simulink model "heli_q8_lab2_part1"  (R2020b)
settings: Solver=ode1  StartTime=0.0  StopTime=inf  FixedStep=0.002  RelTol=1e-3  EnableMultiTasking=on
PostLoadFcn:
  | qc_set_target_type(getConfigSet(bdroot, 'QUARC Default Target Configuration'));
values from neighbouring files (symbols this model uses):
  elev_const = 0.53    [init_heli_3_10_part_4.m]
  F_1 = [K_1(1,1) K_1(1,3) ... (first row only)    [init_heli_3_10_part_4.m]
  Joystick_gain_x = 1    [init_heli_3_10_part_4.m]
  Joystick_gain_y = -1    [init_heli_3_10_part_4.m]
  K_1 = lqr(A,B, Q_lqr, R_lqr)    [init_heli_3_10_part_4.m]
  V_s_0 = 7.77    [init_heli_3_10_part_4.m]
undefined symbols (not defined in the file or in its folder): HIL, qc_get_step_size, sigbuilder_block
libraries: quarc_library x4
settings Model: SimulationMode=external  ExtModeTrigDuration=5000  Creator=Rchan  LastModifiedBy=saavim
settings SolverCC: PositivePriorityOrder=on
settings DataIOCC: LimitDataPoints=on  SaveFormat=Array  SignalLoggingSaveFormat=ModelDataLogs  ReturnWorkspaceOutputs=off
settings OptimizationCC: ExpressionDepthLimit=2147483647  InitFltsAndDblsToZero=on  LifeSpan=inf
settings DebuggingCC: SaveWithParameterizedLinksMsg=none  UnderspecifiedInitializationDetection=Classic  MergeDetectMultiDrivingBlocksExec=none  SolverPrmCheckMsg=warning  MultiTaskDSMMsg=warning  MultiTaskCondExecSysMsg=none  FcnCallInpInsideContextMsg=warning  AllowSymbolicDim=off  StateNameClashWarn=warning  SFUnexpectedBacktrackingDiag=warning  SFNoUnconditionalDefaultTransitionDiag=warning  SFExecutionAtInitializationDiag=none  ArithmeticOperatorsInVariantConditions=warning
settings HardwareCC: ProdBitPerPointer=32  ProdBitPerSizeT=32  ProdBitPerPtrDiffT=32  ProdLargestAtomicFloat=None  ProdIntDivRoundTo=Undefined  ProdEndianess=Unspecified  ProdWordSize=32  ProdHWDeviceType=32-bit Generic
settings ModelReferenceCC: PropagateSignalLabelsOutOfModel=off
settings SFSimCC: SimUseLocalCustomCode=off  CustomCodeUndefinedFunction=UseInterfaceOnly
settings RTWCC: Description=QUARC Win64 Target  SystemTargetFile=quarc_win64.tlc  TemplateMakefile=quarc_default_tmf  RTWUseLocalCustomCode=off
settings CodeAppCC: StateflowObjectComments=on
settings GRTTargetCC: TargetLangStandard=C89/C90 (ANSI)  ParMdlRefBuildCompliant=off  CompOptLevelCompliant=off  CombineOutputUpdateFcns=off  MatFileLogging=off  GRTInterface=on  UseToolchainInfoCompliant=off  ExtMode=on  ExtModeMexFile=quarc_comm
settings ConfigComp: CovMetricSettings=dw  CovSaveCumulativeToWorkspaceVar=on  CovSaveSingleToWorkspaceVar=on  CovExternalEMLEnable=off  CovSFcnEnable=off

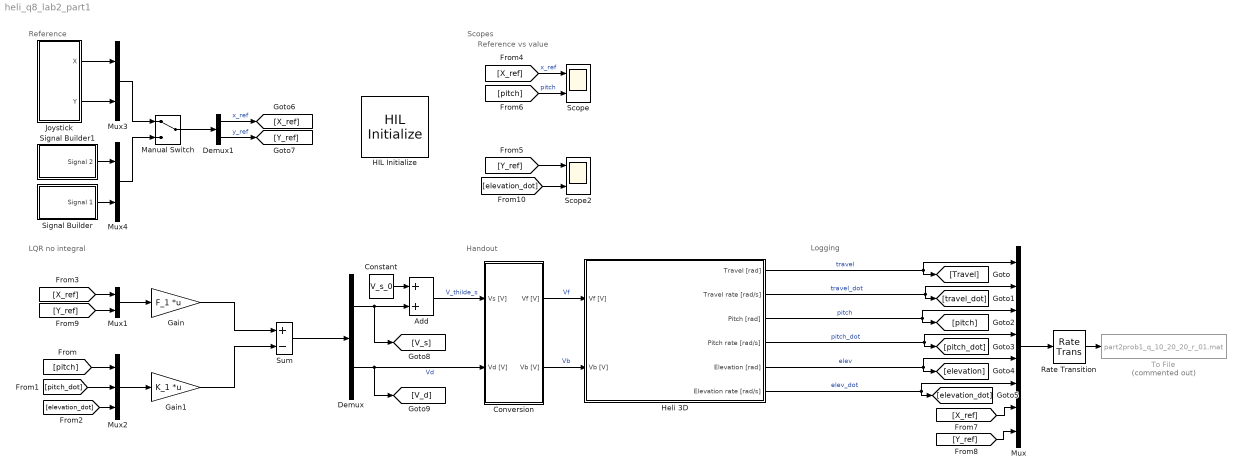
== system heli_q8_lab2_part1 ==
  note: Logging
  note: Handout
  note: Reference
  note: LQR no integral
  note: Scopes
  note: Reference vs value
  Add : Sum
  Constant : Constant  Value=V_s_0
  Conversion : Subsystem
  Demux : Demux  Outputs=2
  Demux1 : Demux  Outputs=2
  Gain : Gain  Gain=F_1  Multiplication=Matrix(K*u)
  Gain1 : Gain  Gain=K_1  Multiplication=Matrix(K*u)
  HIL Initialize : quarc_library/Data Acquisition/Generic/Configuration/HIL Initialize  Priority=-99  object_name=HIL-1  board_type=q8_usb  board_number=0  board_options=update_rate=normal;decimation=1  exclusive=off  active=off  hardware_clocks=[0:2]  clock_modes=[]  initial_clock_frequencies=[]  set_clock_params_at_start=off  set_clock_params_at_switch_in=off  set_clock_frequencies_at_start=off  set_clock_frequencies_at_switch_in=off  analog_input_channels=[0:7]  analog_input_configurations=[]  analog_input_maximums=10  analog_input_minimums=-10  set_analog_input_params_at_start=on  set_analog_input_params_at_switch_in=off  analog_output_channels=[0:7]  analog_output_maximums=10  analog_output_minimums=-10  initial_analog_outputs=[0]  final_analog_outputs=[0]  watchdog_analog_outputs=0  set_analog_output_params_at_start=on  set_analog_output_params_at_switch_in=off  set_analog_outputs_at_start=on  set_analog_outputs_at_switch_in=off  set_analog_outputs_at_terminate=on  set_analog_outputs_at_switch_out=off  set_analog_outputs_on_watchdog=off  digital_input_channels=[]  digital_output_channels=[]  digital_output_configuration=[]  initial_digital_outputs=[1]  final_digital_outputs=[1]  watchdog_digital_outputs=[1]  set_digital_output_params_at_start=off  set_digital_output_params_at_switch_in=off  set_digital_outputs_at_start=on  set_digital_outputs_at_switch_in=off  set_digital_outputs_at_terminate=on  set_digital_outputs_at_switch_out=off  set_digital_outputs_on_watchdog=off  encoder_channels=[0:7]  quadrature=[4]  encoder_filter_frequency=[]  initial_encoder_counts=[0]  set_encoder_params_at_start=on  set_encoder_params_at_switch_in=off  set_encoder_counts_at_start=on  set_encoder_counts_at_switch_in=off  pwm_channels=[0:7]  pwm_modes=0  pwm_frequency=99.532799999999995e6/4095  pwm_configuration=[0]  pwm_alignment=[0]  pwm_polarity=[1]  pwm_leading_deadband=[0]  pwm_trailing_deadband=[0]  initial_pwm_outputs=[0]  final_pwm_outputs=[0]  watchdog_pwm_outputs=[0]  set_pwm_params_at_start=on  set_pwm_params_at_switch_in=off  set_pwm_outputs_at_start=on  set_pwm_outputs_at_switch_in=off  set_pwm_outputs_at_terminate=on  set_pwm_outputs_at_switch_out=off  set_pwm_outputs_on_watchdog=off  other_output_channels=[]  initial_other_outputs=[]  final_other_outputs=[]  watchdog_other_outputs=[]  set_other_outputs_at_start=off  set_other_outputs_at_switch_in=off  set_other_outputs_at_terminate=off  set_other_outputs_at_switch_out=off  set_other_outputs_on_watchdog=off
  Heli 3D : Subsystem
  Joystick : Subsystem
  Manual Switch : ManualSwitch
  Mux : Mux  Inputs=8
  Mux1 : Mux  Inputs=2
  Mux2 : Mux  Inputs=3
  Mux3 : Mux  Inputs=2
  Mux4 : Mux  Inputs=2
  Rate Transition : RateTransition  OutPortSampleTime=0.1
  Scope : Scope  NumInputPorts=2
  Scope2 : Scope  NumInputPorts=2
  Signal Builder : Subsystem  Tag=STV Subsys  LoadFcn=sigbuilder_block('load');  StartFcn=sigbuilder_block('start');  StopFcn=sigbuilder_block('stop');  ClipboardFcn=sigbuilder_block('clipboard');  mask(Sigbuilder block){tuvar=[0:10]}
      mask help: Simulink:masks:SigbuilderBlock_MD
      mask init:
      | if ~strcmp(get_param(bdroot(gcbh),'SimulationStatus'),'stopped') tuvar = sigbuilder_block('maskInit'); end
      settings: CopyFcn=sigbuilder_block('copy');  DeleteFcn=sigbuilder_block('delete');  ModelCloseFcn=sigbuilder_block('modelClose');  PreSaveFcn=sigbuilder_block('preSave');  PauseFcn=sigbuilder_block('pause');  ContinueFcn=sigbuilder_block('continue');  NameChangeFcn=sigbuilder_block('namechange');  OpenFcn=sigbuilder_block('open',[217.5 306 1336.5 574.5 ]);  CloseFcn=sigbuilder_block('close');
      mask Display: plot(0, 0, 100, 100,[2, 2, 32, 32, 2], [68, 8, 8, 68, 68],[32, 2], [38, 38], [32, 19, 2],[53, 60, 44], [32, 17, 17, 2],[16, 16, 31, 31]);txt = getActiveGroup(gcbh);text(2, 100, txt,'verticalAlignment', 'top');
  Signal Builder1 : Subsystem  Tag=STV Subsys  LoadFcn=sigbuilder_block('load');  StartFcn=sigbuilder_block('start');  StopFcn=sigbuilder_block('stop');  ClipboardFcn=sigbuilder_block('clipboard');  mask(Sigbuilder block){tuvar=[0:10]}
      mask help: Simulink:masks:SigbuilderBlock_MD
      mask init:
      | if ~strcmp(get_param(bdroot(gcbh),'SimulationStatus'),'stopped') tuvar = sigbuilder_block('maskInit'); end
      settings: CopyFcn=sigbuilder_block('copy');  DeleteFcn=sigbuilder_block('delete');  ModelCloseFcn=sigbuilder_block('modelClose');  PreSaveFcn=sigbuilder_block('preSave');  PauseFcn=sigbuilder_block('pause');  ContinueFcn=sigbuilder_block('continue');  NameChangeFcn=sigbuilder_block('namechange');  OpenFcn=sigbuilder_block('open',[109.5 258.75 1652.25 670.5 ]);  CloseFcn=sigbuilder_block('close');
      mask Display: plot(0, 0, 100, 100,[2, 2, 32, 32, 2], [68, 8, 8, 68, 68],[32, 2], [38, 38], [32, 19, 2],[53, 60, 44], [32, 17, 17, 2],[16, 16, 31, 31]);txt = getActiveGroup(gcbh);text(2, 100, txt,'verticalAlignment', 'top');
  Sum : Sum  Inputs=+-
  To File : ToFile  Commented=on  Filename=part2prob1_q_10_20_20_r_01.mat
  wires:
  Conversion/2(Vb [V]) -> Heli 3D/2(Vb [V])  "Vb"
  Conversion/1(Vf [V]) -> Heli 3D/1(Vf [V])  "Vf"
  Heli 3D/1(Travel [rad]) -> [Travel], Mux/1  "travel"
  Heli 3D/2(Travel rate [rad/s]) -> [travel_dot], Mux/2  "travel_dot"
  Heli 3D/3(Pitch [rad]) -> [pitch], Mux/3  "pitch"
  Heli 3D/4(Pitch rate [rad/s]) -> [pitch_dot], Mux/4  "pitch_dot"
  Heli 3D/5(Elevation [rad]) -> [elevation], Mux/5  "elev"
  Heli 3D/6(Elevation rate [rad/s]) -> [elevation_dot], Mux/6  "elev_dot"
  [elevation_dot] -> Mux2/3
  Add/1 -> Conversion/1(Vs [V])  "V_thilde_s"
  Mux1/1 -> Gain/1
  Mux2/1 -> Gain1/1
  [pitch_dot] -> Mux2/2
  [pitch] -> Mux2/1
  Gain/1 -> Sum/1
  Gain1/1 -> Sum/2
  Sum/1 -> Demux/1
  Rate Transition/1 -> To File/1
  Mux/1 -> Rate Transition/1
  Demux/2 -> [V_d], Conversion/2(Vd [V])  "Vd"
  Demux/1 -> Add/2, [V_s]
  Constant/1 -> Add/1
  [X_ref] -> Mux/7
  [Y_ref] -> Mux/8
  Joystick/2(Y) -> Mux3/2
  Joystick/1(X) -> Mux3/1
  Mux3/1 -> Manual Switch/1
  Manual Switch/1 -> Demux1/1
  Demux1/1 -> [X_ref]  "x_ref"
  Demux1/2 -> [Y_ref]  "y_ref"
  Signal Builder1/1(Signal 2) -> Mux4/1
  Signal Builder/1(Signal 1) -> Mux4/2
  Mux4/1 -> Manual Switch/2
  [Y_ref] -> Mux1/2
  [X_ref] -> Mux1/1
  [pitch] -> Scope/2  "pitch"
  [elevation_dot] -> Scope2/2
  [Y_ref] -> Scope2/1
  [X_ref] -> Scope/1  "x_ref"

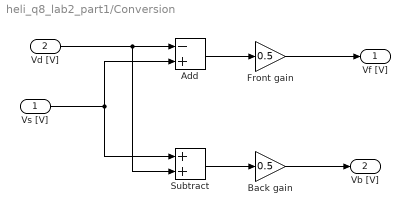
== system heli_q8_lab2_part1/Conversion ==
  Vs [V] : Inport
  Vd [V] : Inport  Port=2
  Add : Sum  Inputs=-+
  Back gain : Gain  Gain=0.5
  Front gain : Gain  Gain=0.5
  Subtract : Sum
  Vf [V] : Outport
  Vb [V] : Outport  Port=2
  wires:
  Vd [V]/1 -> Subtract/2, Add/1
  Vs [V]/1 -> Subtract/1, Add/2
  Subtract/1 -> Back gain/1
  Back gain/1 -> Vb [V]/1
  Add/1 -> Front gain/1
  Front gain/1 -> Vf [V]/1

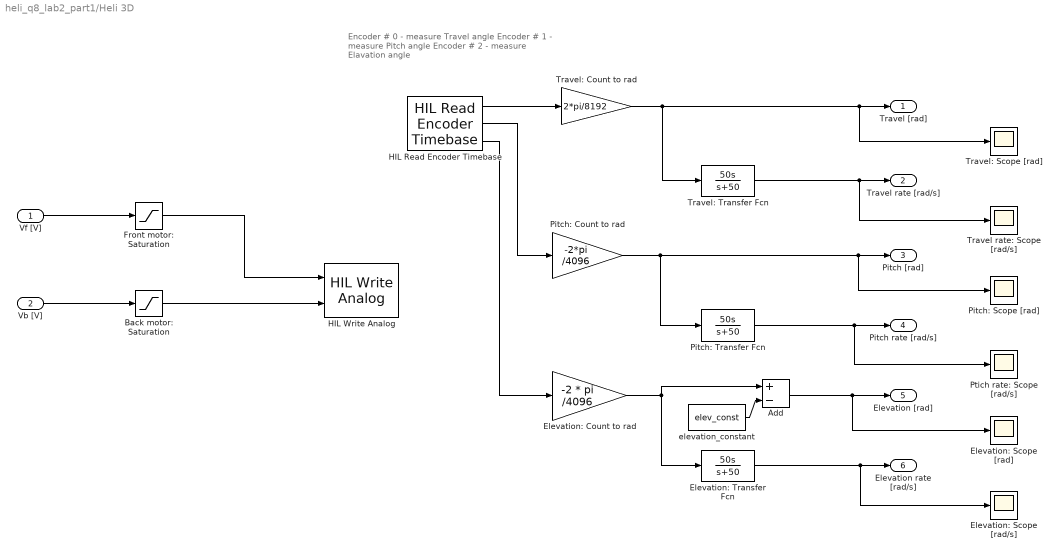
== system heli_q8_lab2_part1/Heli 3D ==
  note: Encoder # 0 - measure Travel angle
      | Encoder # 1 - measure Pitch angle
      | Encoder # 2 - measure Elavation angle
  Vf [V] : Inport
  Vb [V] : Inport  Port=2
  Add : Sum  Inputs=+-
  Back motor: Saturation : Saturate  UpperLimit=5  LowerLimit=-5
  Elevation: Count to rad : Gain  Gain=-2 * pi /4096
  Elevation: Scope [rad/s] : Scope
  Elevation: Scope [rad] : Scope
  Elevation: Transfer Fcn : TransferFcn  Numerator=[50 0]  Denominator=[1 50]
  Front motor: Saturation : Saturate  UpperLimit=5  LowerLimit=-5
  HIL Read Encoder Timebase : quarc_library/Data Acquisition/Generic/Timebases/HIL Read Encoder Timebase  object_name=HIL-1  clock=0  channels=[0:2]  active=on  vector_output=off  data_type_mode=Inherit via back propagation  data_type=double  overflow_mode=Error on overflow  samples_in_buffer=max(ceil(1/qc_get_step_size), 1)
  HIL Write Analog : quarc_library/Data Acquisition/Generic/Immediate I//O/HIL Write Analog  object_name=HIL-1  channels=[0:1]  sample_time=-1  active=off  vector_input=off
  Pitch: Count to rad : Gain  Gain=-2*pi /4096
  Pitch: Scope [rad] : Scope
  Pitch: Transfer Fcn : TransferFcn  Numerator=[50 0]  Denominator=[1 50]
  Ptich rate: Scope [rad/s] : Scope
  Travel rate: Scope [rad/s] : Scope
  Travel: Count to rad : Gain  Gain=2*pi/8192
  Travel: Scope [rad] : Scope
  Travel: Transfer Fcn : TransferFcn  Numerator=[50 0]  Denominator=[1 50]
  elevation_constant : Constant  Value=elev_const
  Travel [rad] : Outport
  Travel rate [rad/s] : Outport  Port=2
  Pitch [rad] : Outport  Port=3
  Pitch rate [rad/s] : Outport  Port=4
  Elevation [rad] : Outport  Port=5
  Elevation rate [rad/s] : Outport  Port=6
  wires:
  HIL Read Encoder Timebase/1 -> Travel: Count to rad/1
  HIL Read Encoder Timebase/2 -> Pitch: Count to rad/1
  HIL Read Encoder Timebase/3 -> Elevation: Count to rad/1
  Travel: Count to rad/1 -> Travel: Scope [rad]/1, Travel [rad]/1, Travel: Transfer Fcn/1
  Travel: Transfer Fcn/1 -> Travel rate: Scope [rad/s]/1, Travel rate [rad/s]/1
  Pitch: Count to rad/1 -> Pitch: Transfer Fcn/1, Pitch: Scope [rad]/1, Pitch [rad]/1
  Pitch: Transfer Fcn/1 -> Ptich rate: Scope [rad/s]/1, Pitch rate [rad/s]/1
  Elevation: Count to rad/1 -> Add/1, Elevation: Transfer Fcn/1
  Elevation: Transfer Fcn/1 -> Elevation: Scope [rad/s]/1, Elevation rate [rad/s]/1
  Vf [V]/1 -> Front motor: Saturation/1
  Vb [V]/1 -> Back motor: Saturation/1
  Front motor: Saturation/1 -> HIL Write Analog/1
  Back motor: Saturation/1 -> HIL Write Analog/2
  elevation_constant/1 -> Add/2
  Add/1 -> Elevation: Scope [rad]/1, Elevation [rad]/1

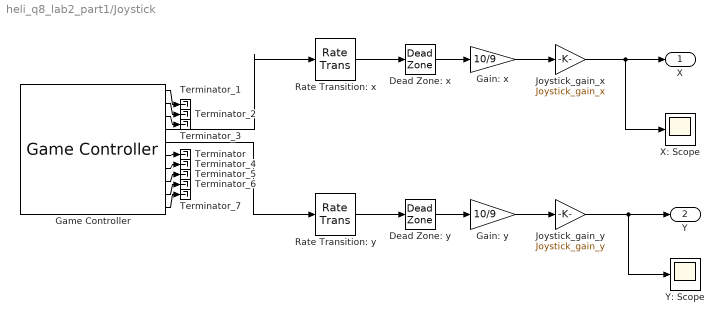
== system heli_q8_lab2_part1/Joystick ==
  Dead Zone: x : DeadZone  LowerValue=-0.1  UpperValue=0.1  SaturateOnIntegerOverflow=on
  Dead Zone: y : DeadZone  LowerValue=-0.1  UpperValue=0.1  SaturateOnIntegerOverflow=on
  Gain: x : Gain  Gain=10/9
  Gain: y : Gain  Gain=10/9
  Game Controller : quarc_library/Devices/Peripherals/Target/Game Controller  controller=1  buffer_size=12  deadzone=[]  saturation=[]  sample_time=max(qc_get_step_size, 0.01)  auto_center=off  enabled=on
      settings: SourceProductName=QUARC Targets
  Joystick_gain_x : Gain  Gain=Joystick_gain_x
  Joystick_gain_y : Gain  Gain=Joystick_gain_y
  Rate Transition: x : RateTransition
  Rate Transition: y : RateTransition
  Terminator : Terminator
  Terminator_{1..7} (7 alike) : Terminator
  X: Scope : Scope
  Y: Scope : Scope
  X : Outport
  Y : Outport  Port=2
  wires:
  Rate Transition: y/1 -> Dead Zone: y/1
  Rate Transition: x/1 -> Dead Zone: x/1
  Game Controller/5 -> Rate Transition: y/1
  Game Controller/4 -> Rate Transition: x/1
  Game Controller/1 -> Terminator_1/1
  Game Controller/2 -> Terminator_2/1
  Game Controller/7 -> Terminator_4/1
  Game Controller/8 -> Terminator_5/1
  Game Controller/9 -> Terminator_6/1
  Game Controller/10 -> Terminator_7/1
  Game Controller/6 -> Terminator/1
  Dead Zone: x/1 -> Gain: x/1
  Dead Zone: y/1 -> Gain: y/1
  Gain: x/1 -> Joystick_gain_x/1
  Gain: y/1 -> Joystick_gain_y/1
  Joystick_gain_x/1 -> X/1, X: Scope/1
  Joystick_gain_y/1 -> Y: Scope/1, Y/1
  Game Controller/3 -> Terminator_3/1

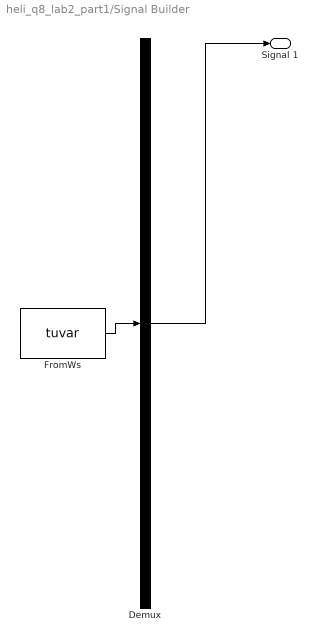
== system heli_q8_lab2_part1/Signal Builder ==
  Demux : Demux  Tag=STV Demux  Outputs=1
      settings: DisplayOption=none
  FromWs : FromWorkspace  Tag=STV FromWs  VariableName=tuvar
      SigBuilderData=|
      | common.afterFinalStr = 'Extrapolate'
      | common.sampleTime = 0
      | dataSet.timeRange = [0 10]
      | dataSet.name = 'Group 1'
      | sbobj.Groups.Name = 'Group 1'
      | sbobj.Groups.Signals.Name = 'Signal 1'
      | sbobj.Groups.Signals.XData = [0 2 2 4 10]
      | sbobj.Groups.Signals.YData = [-0.5 -0.5 0 0 0]
  Signal 1 : Outport  Tag=STV Outport
  wires:
  Demux/1 -> Signal 1/1
  FromWs/1 -> Demux/1

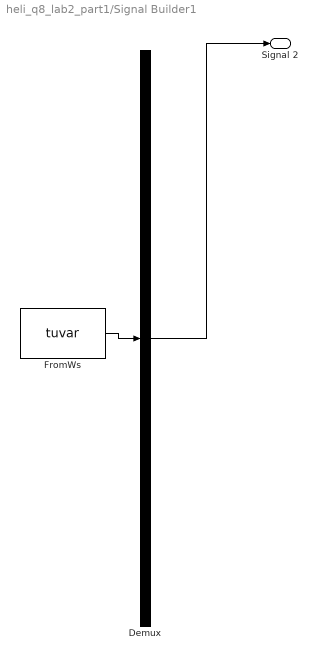
== system heli_q8_lab2_part1/Signal Builder1 ==
  Demux : Demux  Tag=STV Demux  Outputs=1
      settings: DisplayOption=none
  FromWs : FromWorkspace  Tag=STV FromWs  VariableName=tuvar
      SigBuilderData=|
      | common.afterFinalStr = 'Extrapolate'
      | common.sampleTime = 0
      | dataSet.timeRange = [0 60]
      | dataSet.name = 'Group 1'
      | sbobj.Groups.Name = 'Group 1'
      | sbobj.Groups.Signals.Name = 'Signal 2'
      | sbobj.Groups.Signals.XData = [0 9 9 13 13 26 26 30 30 60]
      | sbobj.Groups.Signals.YData = [0 0 0.5 0.5 0 0 -0.5 -0.5 0 0]
      | sbobj.Groups.TimeRange = [0 60]
  Signal 2 : Outport  Tag=STV Outport
  wires:
  Demux/1 -> Signal 2/1
  FromWs/1 -> Demux/1
